simulink model "pack36s9p_21700_model"  (R2026a)
settings: Solver=ode23t  StopTime=600  MaxStep=0.5  AbsTol=1e-4
libraries: fl_lib x3, nesl_utility x3, pack36s9p_21700_lib x1
settings Model: Creator=yashi  LastModifiedBy=yashi

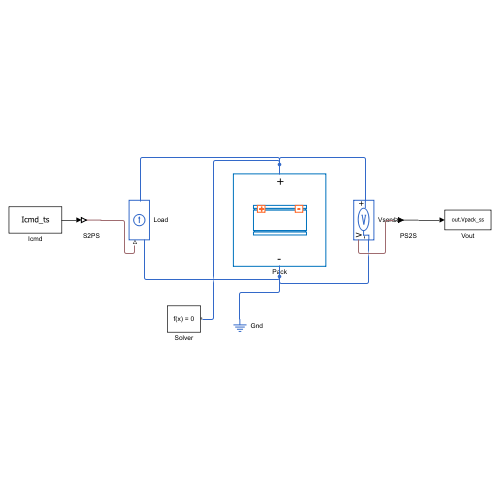
[thumbnail: Simulink's stored preview of the top-level diagram]
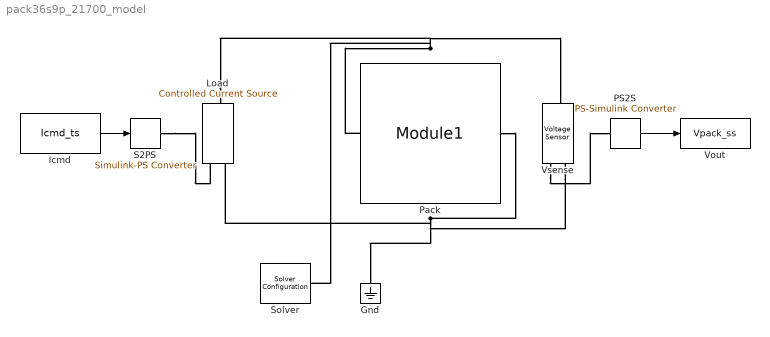
== system pack36s9p_21700_model ==
  Gnd : fl_lib/Electrical/Electrical Elements/Electrical Reference
  Icmd : FromWorkspace  VariableName=Icmd_ts
  Load : fl_lib/Electrical/Electrical Sources/Controlled Current Source
  PS2S : nesl_utility/PS-Simulink Converter  PhysicalDomain=network_engine_domain  SubClassName=ps_output  LeftPortType=input  RightPortType=output  PseudoPeriodic=off  Frequencies=[]  VectorFormat=inherit  Unit=inherit  AffineConversion=off
  Pack : pack36s9p_21700_lib/Module1  BatteryCapacityCell=4.5 A*hr  ExtrapolationMethodCell=simscape.enum.extrapolation.nearest  SOCBreakpointsCell=[0, .1, .25, .5, .75, .9, 1]  TemperatureBreakpointsCell=[278, 293, 313] K  OpenCircuitVoltageThermalCell=[3.49, 3.5, 3.51; 3.55, 3.57, 3.56; 3.62, 3.63, 3.64; 3.71, 3.71, 3.72; 3.91, 3.93, 3.94; 4.07, 4.08, 4.08; 4.19, 4.19, 4.19] V  VoltageRangeCell=[0, inf] V  ResistanceSOCBreakpointsCell=[0, .1, .25, .5, .75, .9, 1]  ResistanceTemperatureBreakpointsCell=[278, 293, 313] K  R0ThermalCell=[.0117, .0085, .009; .011, .0085, .009; .0114, .0087, .0092; .0107, .0082, .0088; .0107, .0083, .0091; .0113, .0085, .0089; .0116, .0085, .0089] Ohm  SimulationTemperatureCell=298.15 K  socCell_specify=off  socCell_priority=High  socCell=0.9  socCell_nominal_specify=off  socCell_nominal_value=1  socCell_nominal_unit=1  batteryVoltage_specify=off  batteryVoltage_priority=None  batteryVoltage=0 V  batteryVoltage_nominal_specify=off  batteryVoltage_nominal_value=1  batteryVoltage_nominal_unit=V  batteryCurrent_specify=off  batteryCurrent_priority=None  batteryCurrent=0 A  batteryCurrent_nominal_specify=off  batteryCurrent_nominal_value=1  batteryCurrent_nominal_unit=A  numCycles_specify=off  numCycles_priority=High  numCycles=0  numCycles_nominal_specify=off  numCycles_nominal_value=1  numCycles_nominal_unit=1  vParallelAssembly_specify=off  vParallelAssembly_priority=None  vParallelAssembly=repmat(0, 36, 1) V  vParallelAssembly_nominal_specify=off  vParallelAssembly_nominal_value=1  vParallelAssembly_nominal_unit=V  socParallelAssembly_specify=off  socParallelAssembly_priority=None  socParallelAssembly=repmat(1, 36, 1)  socParallelAssembly_nominal_specify=off  socParallelAssembly_nominal_value=1  socParallelAssembly_nominal_unit=1
  S2PS : nesl_utility/Simulink-PS Converter  PhysicalDomain=network_engine_domain  SubClassName=ps_input  LeftPortType=input  RightPortType=output  PseudoPeriodic=off  Frequencies=[]  NoiseDistribution=none  NoiseParameters=[]  Unit=1  AffineConversion=off  FilteringAndDerivatives=provide  SimscapeFilterOrder=1  InputFilterTimeConstant=0.001  UdotUserProvided=0
  Solver : nesl_utility/Solver Configuration  PhysicalDomain=network_engine_domain  SubClassName=solver  LeftPortType=input  RightPortType=generic  Tones=[]  Harmonics=[]  SimulateNoise=off  Profile=off  UseLocalSampling=off  EnableSwitchedLinearOptims=on  FrequencyDomain=off  UseCCode=off  RelTol=0.001  AbsTol=0.001  MinStep=1e-09  ToWorkspace=off  RevertToSquareIcSolve=off  NumHomotopyIterations=100  PhasorMode=off  PhasorModeNumHarmonics=1  ConsistencySolver=NEWTON_XTOL_AFTER_FTOL  CanonicalOrdering=CANONICAL  OptimizeIntermediates=OPTIMIZED  IndexReductionMethod=DerivativeReplacement  DoDC=off  ResidualTolerance=1e-09  ConsistencyTolSource=GLOBAL  ConsistencyAbsTol=0.001  ConsistencyRelTol=0.001  ConsistencyTolFactor=0.001  UseLocalSolver=off  LocalSolverChoice=NE_BACKWARD_EULER_ADVANCER  ResolveIndetEquations=on  FunctionEvalNumThread=1  LocalSolverSampleTime=0.001  DoFixedCost=off  MaxNonlinIter=3  MaxModeIter=2  ComputeImpulses=off  ImpulseIterations=2  LinearAlgebra=auto  LinearAlgebraNumThread=0  EquationFormulation=NE_TIME_EF  DelaysMemoryBudget=1024  AutomaticFiltering=on  FilteringTimeConstant=0.001  PartitionStorageMethod=AS_NEEDED  PartitionMemoryBudget=1024  PartitionMethod=ROBUST  MultibodyUseLocalSolver=off  MultibodyLocalSolverChoice=ODE1  MultibodyLocalSolverSampleTime=0.001
  Vout : ToWorkspace  VariableName=Vpack_ss  SaveFormat=Structure With Time  SampleTime=-1
  Vsense : fl_lib/Electrical/Electrical Sensors/Voltage Sensor
  wires:
  Icmd/1 -> S2PS/1
  PS2S/1 -> Vout/1
  connections:
  S2PS/RConn1 -- Load/RConn1
  Vsense/RConn1 -- PS2S/LConn1
  Load/LConn1 -- Pack/LConn1 -- Vsense/LConn1 -- Solver/RConn1
  Load/RConn2 -- Pack/RConn1 -- Vsense/RConn2 -- Gnd/LConn1
